simulink model "pendulum"  (R2025a)
settings: Solver=VariableStepAuto  StartTime=0.0  StopTime=10.0  MaxStep=0.05  RelTol=1e-3
undefined symbols (not defined in the file or in its folder): I
libraries: simulink_extras x2
settings Model: Creator=HP  LastModifiedBy=LaL
settings RTWCC: GPUComputeCapability=3.5

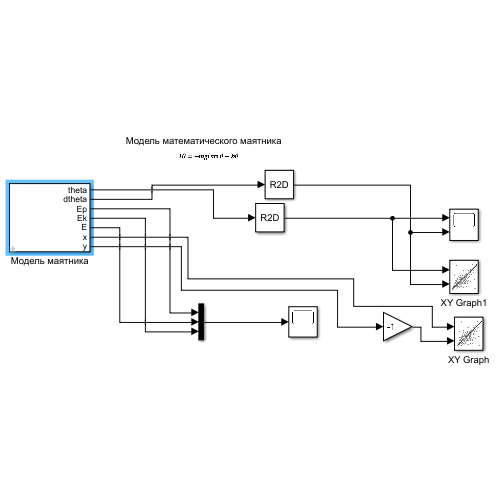
[thumbnail: Simulink's stored preview of the top-level diagram]
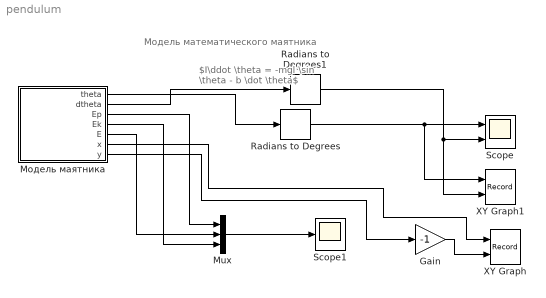
== system pendulum ==
  note: $I\ddot \theta = -mgl \sin \theta - b \dot \theta$
  note: Модель математического маятника
  Gain : Gain  Gain=-1
  Mux : Mux  Inputs=3
  Radians to Degrees : simulink_extras/Transformations/Radians to Degrees
  Radians to Degrees1 : simulink_extras/Transformations/Radians to Degrees
  Scope : Scope  NumInputPorts=2
      settings: ActiveDisplayYMinimum=-26.694018928813971  ActiveDisplayYMaximum=23.652044181418734
  Scope1 : Scope
      settings: ActiveDisplayYMinimum=-0.025150697320047197  ActiveDisplayYMaximum=0.15210845847100571
  XY Graph : Record  NumPorts=2.0  FileSettingsInternal="{\"entries\":[{\"content\":{\"excelSettings\":{\"content\":{},\"type\":\"Streamout.ExcelSettings\"},\"parquetSettings\":{\"content\":{},\"type\":\"Streamout.ParquetSettings\"}},\"type\":\"Streamout.FileSettingStorage\",\"uuid\":\"\"}],\"packageUris\":[\"http:\\/\\/schema.mathworks.com\\/mf0\\/streamout_blocks\\/R2020a\"],\"version\":\"1.0\"}"  FrameSettings=[0, 0]  Layout=[1 1]  SignalsInternal="{\"entries\":[{\"content\":{\"signals\":[{\"content\":{\"blockPath\":[],\"dimensions\":[1],\"domain\":\"\",\"lineColor\":\"#a2142f\",\"plots\":[ 1 ],\"port\":1,\"sid\":[\"\"],\"signalID\":1,\"signalName\":\"Модель маятника:6\"},\"type\":\"RecordBlkView.Signal\",\"uuid\":\"\"},{\"content\":{\"blockPath\":[],\"dimensions\":[1],\"domain\":\"\",\"lineColor\":\"#139fff\",\"plots\":[ 1 ],\"port\":2,\"sid\":[\"\"],\"signalID\":2,\"signalName\":\"Gain\"},\"type\":\"RecordBlkView.Signal\",\"uuid\":\"\"}]},\"type\":\"RecordBlkView.InputSignals\",\"uuid\":\"\"}],\"packageUris\":[\"http:\\/\\/schema.mathworks.com\\/mf0\\/streamout_blocks\\/R2020a\"],\"version\":\"1.0\"}"  VisualizationBindings="{\"xyplotplugin\":{\"info\":[{\"series\":[{\"bindingParametersList\":[{\"parameter\":\"X-Axis\",\"signalID\":1,\"signalName\":\"Модель маятника:6\"},{\"parameter\":\"Y-Axis\",\"signalID\":2,\"signalName\":\"Gain\"}],\"seriesID\":0}],\"subplotID\":1}]}}"  CompatibilityTag=XY  st=-1
  XY Graph1 : Record  NumPorts=2.0  FileSettingsInternal="{\"entries\":[{\"content\":{\"excelSettings\":{\"content\":{},\"type\":\"Streamout.ExcelSettings\"},\"parquetSettings\":{\"content\":{},\"type\":\"Streamout.ParquetSettings\"}},\"type\":\"Streamout.FileSettingStorage\",\"uuid\":\"\"}],\"packageUris\":[\"http:\\/\\/schema.mathworks.com\\/mf0\\/streamout_blocks\\/R2020a\"],\"version\":\"1.0\"}"  FrameSettings=[0, 0]  Layout=[1 1]  SignalsInternal="{\"entries\":[{\"content\":{\"signals\":[{\"content\":{\"blockPath\":[],\"dimensions\":[1],\"domain\":\"\",\"lineColor\":\"#a2142f\",\"plots\":[ 1 ],\"port\":1,\"sid\":[\"\"],\"signalID\":1,\"signalName\":\"Radians\\nto Degrees\"},\"type\":\"RecordBlkView.Signal\",\"uuid\":\"\"},{\"content\":{\"blockPath\":[],\"dimensions\":[1],\"domain\":\"\",\"lineColor\":\"#139fff\",\"plots\":[ 1 ],\"port\":2,\"sid\":[\"\"],\"signalID\":2,\"signalName\":\"Radians\\nto Degrees1\"},\"type\":\"RecordBlkView.Signal\",\"uuid\":\"\"}]},\"type\":\"RecordBlkView.InputSignals\",\"uuid\":\"\"}],\"packageUris\":[\"http:\\/\\/schema.mathworks.com\\/mf0\\/streamout_blocks\\/R2020a\"],\"version\":\"1.0\"}"  VisualizationBindings="{\"xyplotplugin\":{\"info\":[{\"series\":[{\"bindingParametersList\":[{\"parameter\":\"X-Axis\",\"signalID\":1,\"signalName\":\"Radians\\nto Degrees\"},{\"parameter\":\"Y-Axis\",\"signalID\":2,\"signalName\":\"Radians\\nto Degrees1\"}],\"seriesID\":0}],\"subplotID\":1}]}}"  CompatibilityTag=XY  st=-1
  Модель маятника : Subsystem  mask{g=9.815, m=1, l=1, b=0.3, startDegree=0.13}
      mask prompts: g "Гравитация(м/с^2)"; m "Масса груза(кг)"; l "Длина маятника(м)"; b "Декримент затухания"; startDegree "Начальный угол отклонения маятника(рад)"
  wires:
  Модель маятника/1(theta) -> Radians to Degrees/1
  Модель маятника/2(dtheta) -> Radians to Degrees1/1
  Radians to Degrees/1 -> XY Graph1/1, Scope/1
  Модель маятника/3(Ep) -> Mux/1
  Модель маятника/4(Ek) -> Mux/3
  Модель маятника/5(E) -> Mux/2
  Mux/1 -> Scope1/1
  Модель маятника/7(y) -> Gain/1
  Модель маятника/6(x) -> XY Graph/1
  Radians to Degrees1/1 -> XY Graph1/2, Scope/2
  Gain/1 -> XY Graph/2

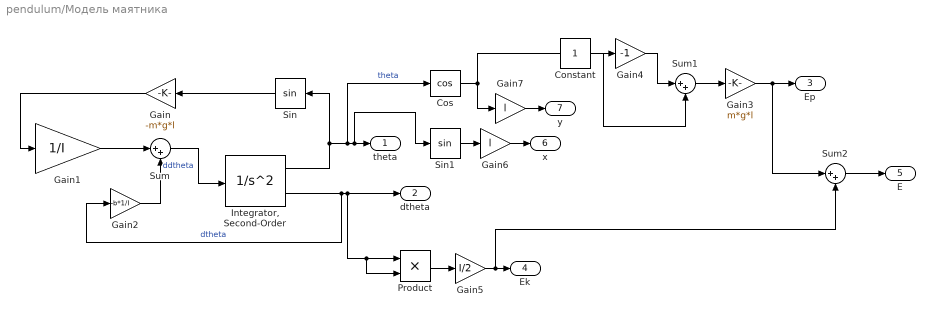
== system pendulum/Модель маятника ==
  Constant : Constant
  Cos : Trigonometry  Operator=cos
  Gain : Gain  Gain=-m*g*l
  Gain1 : Gain  Gain=1/I
  Gain2 : Gain  Gain=-b*1/I
  Gain3 : Gain  Gain=m*g*l
  Gain4 : Gain  Gain=-1
  Gain5 : Gain  Gain=I/2
  Gain6 : Gain  Gain=l
  Gain7 : Gain  Gain=l
  "Integrator, Second-Order" : SecondOrderIntegrator  ICX=startDegree
  Product : Product
  Sin : Trigonometry
  Sin1 : Trigonometry
  Sum : Sum  Inputs=|++
  Sum1 : Sum  Inputs=|++
  Sum2 : Sum  Inputs=|++
  theta : Outport
  dtheta : Outport  Port=2
  Ep : Outport  Port=3
  Ek : Outport  Port=4
  E : Outport  Port=5
  x : Outport  Port=6
  y : Outport  Port=7
  wires:
  Sin/1 -> Gain/1
  Gain/1 -> Gain1/1
  "Integrator, Second-Order"/1 -> Cos/1, Sin1/1, theta/1, Sin/1  "theta"
  Gain1/1 -> Sum/1
  "Integrator, Second-Order"/2 -> Gain2/1, Product/2, Product/1, dtheta/1  "dtheta"
  Sum/1 -> "Integrator, Second-Order"/1  "ddtheta"
  Gain2/1 -> Sum/2
  Cos/1 -> Gain7/1, Gain4/1
  Gain4/1 -> Sum1/1
  Constant/1 -> Sum1/2
  Sum1/1 -> Gain3/1
  Gain3/1 -> Sum2/1, Ep/1
  Product/1 -> Gain5/1
  Gain5/1 -> Sum2/2, Ek/1
  Sum2/1 -> E/1
  Sin1/1 -> Gain6/1
  Gain6/1 -> x/1
  Gain7/1 -> y/1
